simulink model "multirateEKFExample2"  (R2019a)
settings: Solver=VariableStepAuto  StartTime=0.0  StopTime=10  RelTol=1e-3
libraries: sharedTrackingLibrary x1
settings Model: Creator=The MathWorks, Inc.  LastModifiedBy=ditt_aj
settings DataIOCC: ReturnWorkspaceOutputs=off
settings DebuggingCC: PregeneratedLibrarySubsystemCodeDiagnostic=none  ArithmeticOperatorsInVariantConditions=warning
settings SFSimCC: SimUseLocalCustomCode=off
settings RTWCC: RTWUseLocalCustomCode=off
settings CodeAppCC: StateflowObjectComments=on

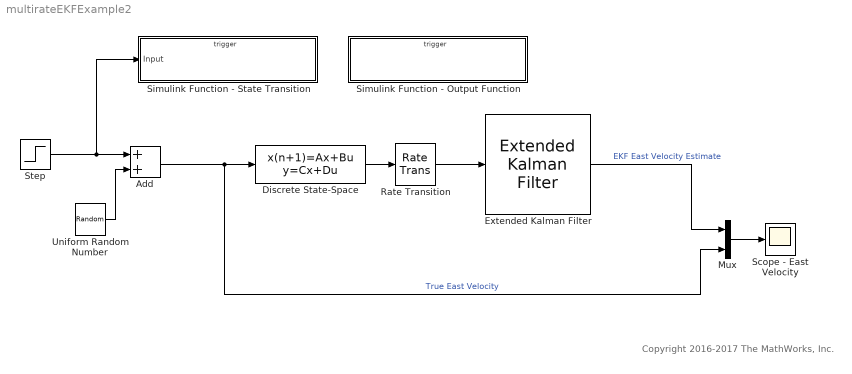
== system multirateEKFExample2 ==
  note: Copyright 2016-2017 The MathWorks, Inc.
  Add : Sum
  Discrete State-Space : DiscreteStateSpace  A=0.1  B=0.9  D=0  SampleTime=-1
  Extended Kalman Filter : sharedTrackingLibrary/Extended Kalman Filter  StateTransitionFcn=stateTransitionFcn  HasStateTransitionJacobianFcn=off  StateTransitionJacobianFcn=stateTransitionJacobianFcn  HasAdditiveProcessNoise=Additive  ProcessNoise=1  HasTimeVaryingProcessNoise=off  HasStateTransitionFcnExtraArgument=0  InitialState=0  InitialStateCovariance=10  MeasurementFcn1=outputFcn  HasMeasurementJacobianFcn1=off  HasMeasurementEnablePort1=off  HasAdditiveMeasurementNoise1=Additive  MeasurementNoise1=0.1  HasTimeVaryingMeasurementNoise1=off  HasMeasurementFcnExtraArgument1=0  MeasurementFcn2=gpsMeasurementFcn  HasMeasurementJacobianFcn2=off  HasMeasurementEnablePort2=off  HasAdditiveMeasurementNoise2=Additive  MeasurementNoise2=[100 0; 0 100]  HasTimeVaryingMeasurementNoise2=off  HasMeasurementFcnExtraArgument2=0  MeasurementFcn3=myMeasurementFcn  HasMeasurementJacobianFcn3=off  HasMeasurementEnablePort3=off  HasAdditiveMeasurementNoise3=Additive  MeasurementNoise3=1  HasTimeVaryingMeasurementNoise3=off  HasMeasurementFcnExtraArgument3=0  MeasurementFcn4=myMeasurementFcn  HasMeasurementJacobianFcn4=off  HasMeasurementEnablePort4=off  HasAdditiveMeasurementNoise4=Additive  MeasurementNoise4=1  HasTimeVaryingMeasurementNoise4=off  HasMeasurementFcnExtraArgument4=0  MeasurementFcn5=myMeasurementFcn  HasMeasurementJacobianFcn5=off  HasMeasurementEnablePort5=off  HasAdditiveMeasurementNoise5=Additive  MeasurementNoise5=1  HasTimeVaryingMeasurementNoise5=off  HasMeasurementFcnExtraArgument5=0  EnableMultirate=on  StateTransitionFcnSampleTime=0.05  MeasurementFcn1SampleTime=0.05  MeasurementFcn2SampleTime=1  MeasurementFcn3SampleTime=-1  MeasurementFcn4SampleTime=-1  MeasurementFcn5SampleTime=-1  UseCurrentEstimator=on  OutputStateCovariance=off  DataType=double  SampleTime=1  NumberOfMeasurements=1
      settings: SourceProductName=Control System Toolbox  SourceProductBaseCode=CT
  Mux : Mux  Inputs=2
  Rate Transition : RateTransition
  Scope - East Velocity : Scope
  Simulink Function - Output Function : Subsystem  TreatAsAtomicUnit=on
  Simulink Function - State Transition : Subsystem  TreatAsAtomicUnit=on
  Step : Step  SampleTime=0
  Uniform Random Number : UniformRandomNumber
  wires:
  Discrete State-Space/1 -> Rate Transition/1
  Mux/1 -> Scope - East Velocity/1
  Add/1 -> Mux/2, Discrete State-Space/1  "True East Velocity"
  Extended Kalman Filter/1 -> Mux/1  "EKF East Velocity Estimate"
  Step/1 -> Simulink Function - State Transition/1(Input), Add/1
  Uniform Random Number/1 -> Add/2
  Rate Transition/1 -> Extended Kalman Filter/1

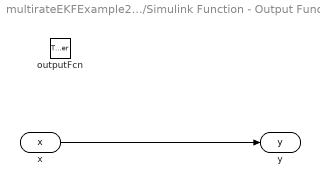
== system multirateEKFExample2/Simulink Function - Output Function ==
  outputFcn : TriggerPort  TriggerType=function-call  IsSimulinkFunction=on  FunctionName=outputFcn  VariantControl=Variant
  x : ArgIn  DisableCoverage=on  ArgumentName=x
  y : ArgOut  DisableCoverage=on  ArgumentName=y
  wires:
  x/1 -> y/1

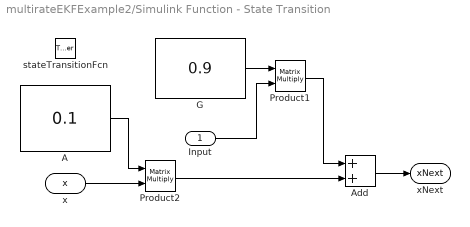
== system multirateEKFExample2/Simulink Function - State Transition ==
  Input : Inport
  stateTransitionFcn : TriggerPort  TriggerType=function-call  IsSimulinkFunction=on  FunctionName=stateTransitionFcn  VariantControl=Variant
  A : Constant  Value=0.1
  Add : Sum
  G : Constant  Value=0.9
  Product1 : Product  Multiplication=Matrix(*)
  Product2 : Product  Multiplication=Matrix(*)
  x : ArgIn  DisableCoverage=on  ArgumentName=x
  xNext : ArgOut  DisableCoverage=on  ArgumentName=xNext
  wires:
  x/1 -> Product2/2
  A/1 -> Product2/1
  Product2/1 -> Add/2
  G/1 -> Product1/1
  Input/1 -> Product1/2
  Product1/1 -> Add/1
  Add/1 -> xNext/1
